simulink model "task1"  (R2024b)
settings: Solver=VariableStepAuto  StartTime=0.0  StopTime=10.0  RelTol=1e-3
settings Model: Creator=33657  LastModifiedBy=33657

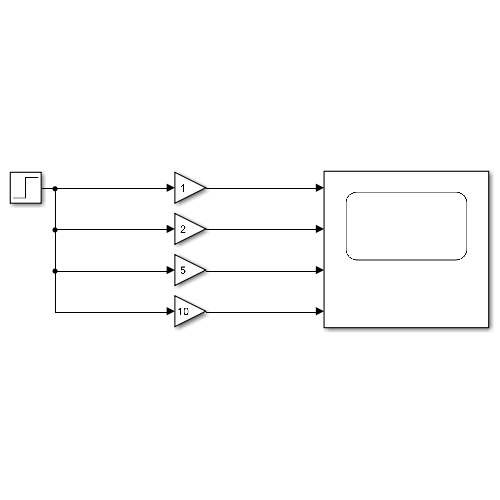
[thumbnail: Simulink's stored preview of the top-level diagram]
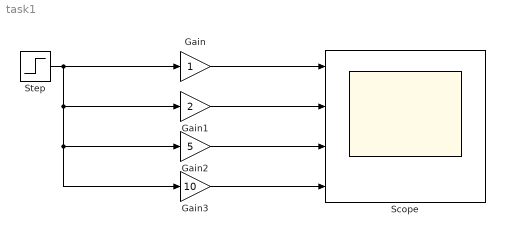
== system task1 ==
  Gain : Gain
  Gain1 : Gain  Gain=2
  Gain2 : Gain  Gain=5
  Gain3 : Gain  Gain=10
  Scope : Scope  NumInputPorts=4
  Step : Step  SampleTime=0
  wires:
  Step/1 -> Gain3/1, Gain2/1, Gain1/1, Gain/1
  Gain/1 -> Scope/1
  Gain3/1 -> Scope/4
  Gain2/1 -> Scope/3
  Gain1/1 -> Scope/2
